simulink model "two_area_agc"  (R2024b)
settings: Solver=VariableStepAuto  StartTime=0.0  StopTime=50  RelTol=1e-3
settings Model: Creator=HP  LastModifiedBy=faisa
settings SolverCC: AlgebraicLoopSolver=TrustRegion
settings DataIOCC: ReturnWorkspaceOutputs=off
settings DebuggingCC: UnconnectedInputMsg=warning  UnconnectedOutputMsg=warning  UnconnectedLineMsg=warning  ArithmeticOperatorsInVariantConditions=warning
settings ModelReferenceCC: EnableRefExpFcnMdlSchedulingChecks=on
settings SFSimCC: SimUseLocalCustomCode=off  CustomCodeUndefinedFunction=UseInterfaceOnly
settings RTWCC: RTWUseLocalCustomCode=off  GPUComputeCapability=3.5
settings CodeAppCC: StateflowObjectComments=on

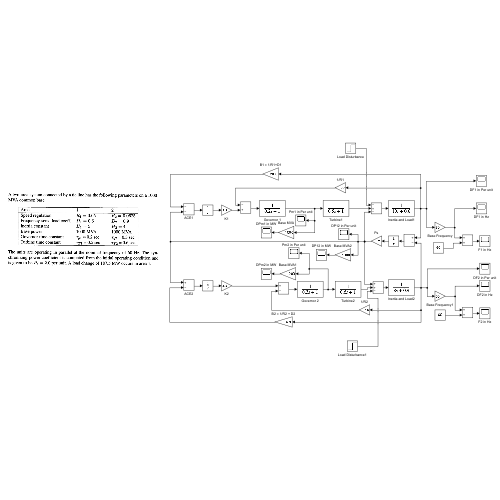
[thumbnail: Simulink's stored preview of the top-level diagram]
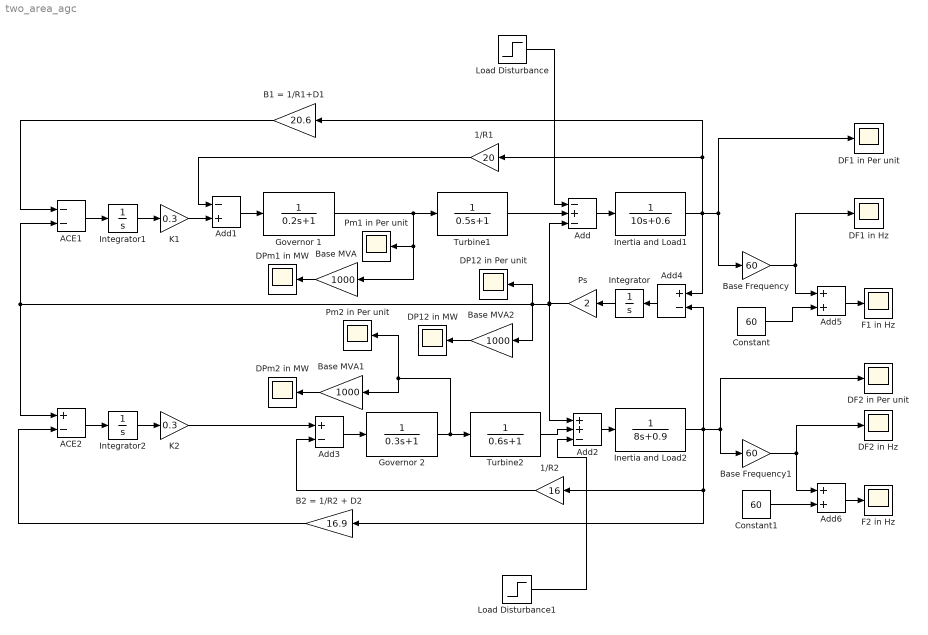
== system two_area_agc ==
  1/R1 : Gain  Gain=20
  1/R2 : Gain  Gain=16
  ACE1 : Sum  Inputs=--
  ACE2 : Sum  Inputs=+-
  Add : Sum  Inputs=-+-
  Add1 : Sum  Inputs=-+
  Add2 : Sum  Inputs=++-
  Add3 : Sum  Inputs=+-
  Add4 : Sum  Inputs=+-
  Add5 : Sum
  Add6 : Sum
  B1 = 1/R1+D1 : Gain  Gain=20.6
  B2 = 1/R2 + D2 : Gain  Gain=16.9
  Base Frequency : Gain  Gain=60
  Base Frequency1 : Gain  Gain=60
  Base MVA : Gain  Gain=1000
  Base MVA1 : Gain  Gain=1000
  Base MVA2 : Gain  Gain=1000
  Constant : Constant  Value=60
  Constant1 : Constant  Value=60
  DF1 in Hz : Scope
  DF1 in Per unit : Scope
  DF2 in Hz : Scope
  DF2 in Per unit : Scope
  DP12 in MW : Scope
  DP12 in Per unit : Scope
  DPm1 in MW : Scope
  DPm2 in MW : Scope
  F1 in Hz : Scope
  F2 in Hz : Scope
  Governor 1 : TransferFcn  Denominator=[0.2 1]
  Governor 2 : TransferFcn  Denominator=[0.3 1]
  Inertia and Load1 : TransferFcn  Denominator=[10 0.6]
  Inertia and Load2 : TransferFcn  Denominator=[8 0.9]
  Integrator : Integrator
  Integrator1 : Integrator
  Integrator2 : Integrator
  K1 : Gain  Gain=0.3
  K2 : Gain  Gain=0.3
  Load Disturbance : Step  Time=100  Before=0.1875  After=0.1875  SampleTime=0
  Load Disturbance1 : Step  Time=100  After=0  SampleTime=0
  Pm1 in Per unit : Scope
  Pm2 in Per unit : Scope
  Ps : Gain  Gain=2
  Turbine1 : TransferFcn  Denominator=[0.5 1]
  Turbine2 : TransferFcn  Denominator=[0.6 1]
  wires:
  Add/1 -> Inertia and Load1/1
  Turbine1/1 -> Add/2
  Governor 1/1 -> Pm1 in Per unit/1, Base MVA/1, Turbine1/1
  Add1/1 -> Governor 1/1
  1/R1/1 -> Add1/1
  Add2/1 -> Inertia and Load2/1
  Turbine2/1 -> Add2/2
  Add3/1 -> Governor 2/1
  Governor 2/1 -> Pm2 in Per unit/1, Base MVA1/1, Turbine2/1
  Add4/1 -> Integrator/1
  Integrator/1 -> Ps/1
  Ps/1 -> Add/3, DP12 in Per unit/1, ACE2/1, ACE1/2, Base MVA2/1, Add2/1
  Load Disturbance/1 -> Add/1
  Base Frequency/1 -> DF1 in Hz/1, Add5/1
  Base Frequency1/1 -> DF2 in Hz/1, Add6/1
  Constant/1 -> Add5/2
  Add5/1 -> F1 in Hz/1
  Constant1/1 -> Add6/2
  Add6/1 -> F2 in Hz/1
  Base MVA/1 -> DPm1 in MW/1
  Base MVA1/1 -> DPm2 in MW/1
  Base MVA2/1 -> DP12 in MW/1
  B1 = 1/R1+D1/1 -> ACE1/1
  Inertia and Load1/1 -> Base Frequency/1, DF1 in Per unit/1, Add4/1, B1 = 1/R1+D1/1, 1/R1/1
  ACE1/1 -> Integrator1/1
  Integrator1/1 -> K1/1
  K1/1 -> Add1/2
  Inertia and Load2/1 -> DF2 in Per unit/1, Base Frequency1/1, B2 = 1/R2 + D2/1, 1/R2/1, Add4/2
  B2 = 1/R2 + D2/1 -> ACE2/2
  ACE2/1 -> Integrator2/1
  Integrator2/1 -> K2/1
  K2/1 -> Add3/1
  1/R2/1 -> Add3/2
  Load Disturbance1/1 -> Add2/3
